simulink model "Mophong"  (R2024a)
settings: Solver=ode3  StartTime=0.0  StopTime=10  FixedStep=0.01  RelTol=1e-3
values from neighbouring files (symbols this model uses):
  A = [0,                                                                                                                                                                                                                                                                1,                                                                                                                                            ...(+395 chars)    [CacFunctionTrongSimulink_LQR.m]
  B = [                                                                                                                                                                                                                   0,                                                                                                                                                                                           ...(+27 chars)    [CacFunctionTrongSimulink_LQR.m]
  C = [1 0 0 0 0 0 ... (first row only)    [CacFunctionTrongSimulink_LQR.m]
  x1_init = 0.003    [CacFunctionTrongSimulink_LQR.m]
  x2_init = -0.0012    [CacFunctionTrongSimulink_LQR.m]
  x4_init = 0.002    [CacFunctionTrongSimulink_LQR.m]
  x5_init = -0.002    [CacFunctionTrongSimulink_LQR.m]
  x7_init = 0.002    [CacFunctionTrongSimulink_LQR.m]
  x8_init = -0.0014    [CacFunctionTrongSimulink_LQR.m]
undefined symbols (not defined in the file or in its folder): K, Lk
libraries: simulink x3
settings Model: Creator=nguye  LastModifiedBy=HP

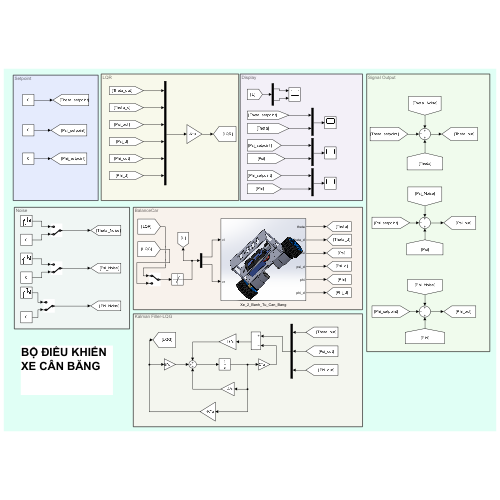
[thumbnail: Simulink's stored preview of the top-level diagram]
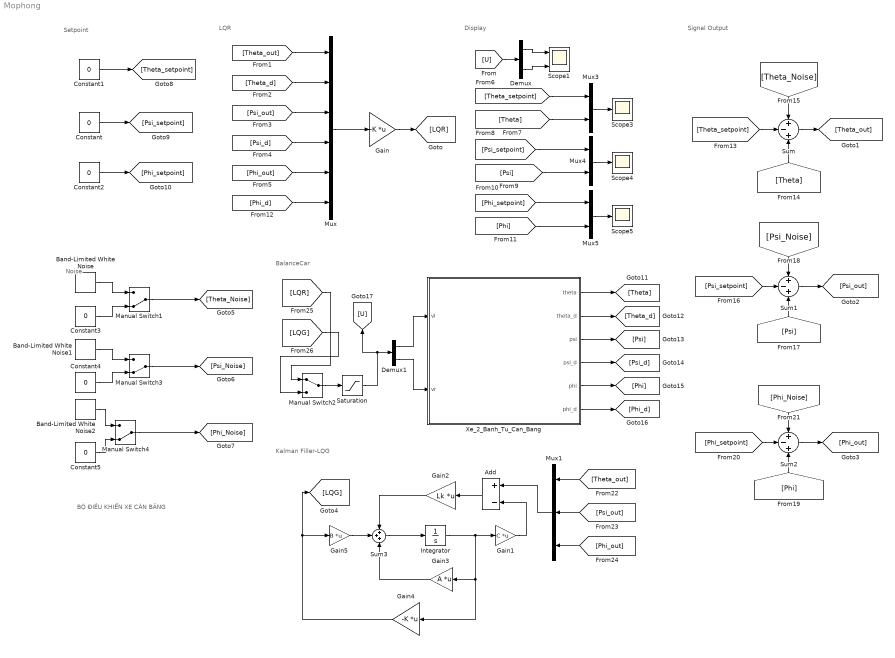
== system Mophong ==
  note: BỘ ĐIỀU KHIỂN XE CÂN BĂNG
  note: BalanceCar
  note: Setpoint
  note: LQR
  note: Display
  note: Signal Output
  note: Kalman Filler-LQG
  note: Noise
  Add : Sum  Inputs=+-
  Band-Limited White Noise : simulink/Sources/Band-Limited White Noise  Cov=[ 0.0001]  Ts=0.01  seed=[23341]
  Band-Limited White Noise1 : simulink/Sources/Band-Limited White Noise  Cov=[0.0000001]  Ts=0.01  seed=[23341]
  Band-Limited White Noise2 : simulink/Sources/Band-Limited White Noise  Cov=[0.00001]  Ts=0.01  seed=[23341]
  Constant{,1..5} (6 alike) : Constant  Value=0
  Demux : Demux  Outputs=2
  Demux1 : Demux  Outputs=2
  Gain : Gain  Gain=-K  Multiplication=Matrix(K*u)
  Gain1 : Gain  Gain=C  Multiplication=Matrix(K*u)
  Gain2 : Gain  Gain=Lk  Multiplication=Matrix(K*u)
  Gain3 : Gain  Gain=A  Multiplication=Matrix(K*u)
  Gain4 : Gain  Gain=-K  Multiplication=Matrix(K*u)
  Gain5 : Gain  Gain=B  Multiplication=Matrix(K*u)
  Integrator : Integrator
  Manual Switch1 : ManualSwitch  CurrentSetting=0
  Manual Switch2 : ManualSwitch
  Manual Switch3 : ManualSwitch  CurrentSetting=0
  Manual Switch4 : ManualSwitch  CurrentSetting=0
  Mux : Mux  Inputs=6
  Mux1 : Mux  Inputs=3
  Mux3 : Mux  Inputs=2
  Mux4 : Mux  Inputs=2
  Mux5 : Mux  Inputs=2
  Saturation : Saturate  UpperLimit=255  LowerLimit=-255
  Scope1 : Scope  NumInputPorts=2
  Scope3 : Scope
  Scope4 : Scope
  Scope5 : Scope
  Sum : Sum  Inputs=+-+
  Sum1 : Sum  Inputs=+-+
  Sum2 : Sum  Inputs=+-+
  Sum3 : Sum  Inputs=+++
  Xe_2_Banh_Tu_Can_Bang : Subsystem
      mask Display: image('BalanceCar.png');
  wires:
  Mux4/1 -> Scope4/1
  Mux3/1 -> Scope3/1
  [Phi] -> Mux5/2
  [Phi_setpoint] -> Mux5/1
  [Psi] -> Mux4/2
  [Psi_setpoint] -> Mux4/1
  [Theta] -> Mux3/2
  [U] -> Demux/1
  Demux/1 -> Scope1/1
  Demux/2 -> Scope1/2
  [Theta_out] -> Mux/1
  [Theta_d] -> Mux/2
  [Psi_out] -> Mux/3
  [Psi_d] -> Mux/4
  [Phi_out] -> Mux/5
  [Phi_d] -> Mux/6
  Mux/1 -> Gain/1
  Gain/1 -> [LQR]
  [Theta_Noise] -> Sum/1
  Sum/1 -> [Theta_out]
  Sum1/1 -> [Psi_out]
  [Psi_Noise] -> Sum1/1
  [Phi_Noise] -> Sum2/1
  Sum2/1 -> [Phi_out]
  [Theta_out] -> Mux1/1
  [Psi_out] -> Mux1/2
  Mux1/1 -> Add/1
  Add/1 -> Gain2/1
  Sum3/1 -> Integrator/1
  Gain3/1 -> Sum3/3
  Gain5/1 -> Sum3/2
  Gain2/1 -> Sum3/1
  Constant2/1 -> [Phi_setpoint]
  Constant1/1 -> [Theta_setpoint]
  Constant/1 -> [Psi_setpoint]
  [LQR] -> Manual Switch2/1
  [LQG] -> Manual Switch2/2
  Integrator/1 -> Gain1/1, Gain4/1, Gain3/1
  Xe_2_Banh_Tu_Can_Bang/1(theta) -> [Theta]
  Xe_2_Banh_Tu_Can_Bang/2(theta_d) -> [Theta_d]
  Xe_2_Banh_Tu_Can_Bang/3(psi) -> [Psi]
  Xe_2_Banh_Tu_Can_Bang/4(psi_d) -> [Psi_d]
  Xe_2_Banh_Tu_Can_Bang/5(phi) -> [Phi]
  Xe_2_Banh_Tu_Can_Bang/6(phi_d) -> [Phi_d]
  Demux1/1 -> Xe_2_Banh_Tu_Can_Bang/1(vl)
  Demux1/2 -> Xe_2_Banh_Tu_Can_Bang/2(vr)
  Mux5/1 -> Scope5/1
  [Phi_out] -> Mux1/3
  Gain4/1 -> [LQG], Gain5/1
  Band-Limited White Noise/1 -> Manual Switch1/1
  Manual Switch1/1 -> [Theta_Noise]
  Constant3/1 -> Manual Switch1/2
  Band-Limited White Noise1/1 -> Manual Switch3/1
  Constant4/1 -> Manual Switch3/2
  Manual Switch3/1 -> [Psi_Noise]
  Band-Limited White Noise2/1 -> Manual Switch4/1
  Manual Switch4/1 -> [Phi_Noise]
  Constant5/1 -> Manual Switch4/2
  Gain1/1 -> Add/2
  [Theta_setpoint] -> Mux3/1
  Manual Switch2/1 -> Saturation/1
  Saturation/1 -> Demux1/1, [U]
  [Theta] -> Sum/3
  [Theta_setpoint] -> Sum/2
  [Psi] -> Sum1/3
  [Psi_setpoint] -> Sum1/2
  [Phi] -> Sum2/3
  [Phi_setpoint] -> Sum2/2

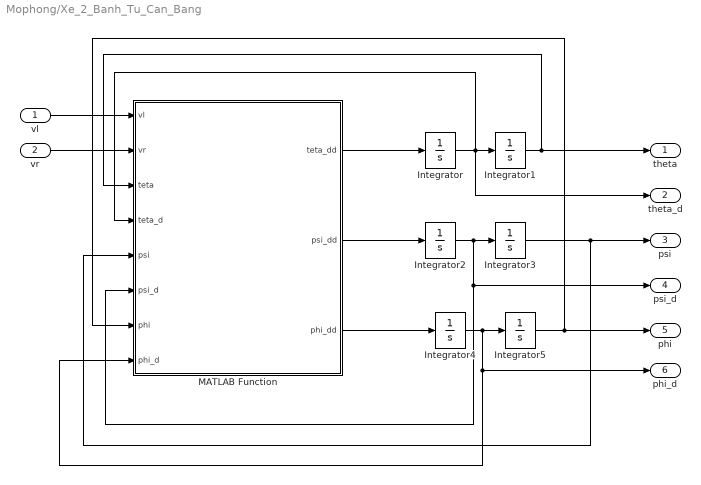
== system Mophong/Xe_2_Banh_Tu_Can_Bang ==
  vl : Inport
  vr : Inport  Port=2
  Integrator : Integrator  InitialCondition=x2_init
  Integrator1 : Integrator  InitialCondition=x1_init
  Integrator2 : Integrator  InitialCondition=x5_init
  Integrator3 : Integrator  InitialCondition=x4_init
  Integrator4 : Integrator  InitialCondition=x8_init
  Integrator5 : Integrator  InitialCondition=x7_init
  MATLAB Function : MATLAB Function  TreatAsAtomicUnit=on
  theta : Outport
  theta_d : Outport  Port=2
  psi : Outport  Port=3
  psi_d : Outport  Port=4
  phi : Outport  Port=5
  phi_d : Outport  Port=6
  wires:
  Integrator/1 -> MATLAB Function/4(teta_d), Integrator1/1, theta_d/1
  Integrator1/1 -> MATLAB Function/3(teta), theta/1
  MATLAB Function/1(teta_dd) -> Integrator/1
  Integrator3/1 -> MATLAB Function/5(psi), psi/1
  Integrator2/1 -> MATLAB Function/6(psi_d), psi_d/1, Integrator3/1
  MATLAB Function/2(psi_dd) -> Integrator2/1
  Integrator5/1 -> MATLAB Function/7(phi), phi/1
  Integrator4/1 -> MATLAB Function/8(phi_d), phi_d/1, Integrator5/1
  MATLAB Function/3(phi_dd) -> Integrator4/1
  vr/1 -> MATLAB Function/2(vr)
  vl/1 -> MATLAB Function/1(vl)

== matlab function Mophong/Xe_2_Banh_Tu_Can_Bang/MATLAB Function ==
  data: vl input; teta_dd output; vr input; teta input; teta_d input; psi input; psi_d input; phi input; phi_d input; psi_dd output; phi_dd output
function [teta_dd,psi_dd,phi_dd] = fcn(vl,vr,teta,teta_d,psi,psi_d,phi,phi_d)

%% Thông số hệ thống xe 2 bánh tự cân bằng dùng LQR
m = 0.033; %Khoi luong banh xe
M = 0.818; %Khoi luong robot
R = 0.0325; %Ban kinh ban xe
W = 0.15; %Chieu dai robot
D = 0.07; %Chieu rong robot
H = 0.095; %Chieu cao robot
L = 0.06; %khoang cach tu trong tam den truc banh xe
fw = 0.18; %He so ma sat giua banh xe voi mat phang
fm = 0.002; %he so ma sat giua dong co va robot
Jm = 0.01; %moment quan tinh cua dong co
Jw = m*R^2/2;
J_psi = 2*M*L^2/3;
J_phi = M*(W^2+D^2)/12;
Rm = 40; %Dien tro dong co DC
Kb = 0.327; %he so emf cua dong co
Kt = 0.5; %Momen xoan cua dong co DC
n = 30; %Ty so giam toc
g = 9.81; %Gia toc trong truong
alpha = (n*Kt)/Rm; beta=((n*Kt*Kb)/Rm)+fm; a =alpha;
T=0.01;

teta_dd = (J_psi*a*vl + J_psi*a*vr - 2*J_psi*beta*teta_d + 2*J_psi*beta*psi_d - 2*J_psi*fw*teta_d + L^2*M*a*vl + L^2*M*a*vr - 2*L^2*M*beta*teta_d + 2*L^2*M*beta*psi_d - 2*L^2*M*fw*teta_d - 4*Jm*fw*n^2*teta_d + L^3*M^2*R*psi_d^2*sin(psi) - 2*L*M*R*beta*teta_d*cos(psi) + 2*L*M*R*beta*psi_d*cos(psi) - L^3*M^2*R*phi_d^2*cos(psi)^2*sin(psi) - L^2*M^2*R*g*cos(psi)*sin(psi) + J_psi*L*M*R*psi_d^2*sin(psi) + 2*Jm*L*M*g*n^2*sin(psi) + L*M*R*a*vl*cos(psi) + L*M*R*a*vr*cos(psi) + 2*Jm*L^2*M*n^2*phi_d^2*cos(psi)*sin(psi) + 2*Jm*L*M*R*n^2*psi_d^2*sin(psi))/(2*J_psi*Jw + L^2*M^2*R^2 + 2*Jw*L^2*M + J_psi*M*R^2 + 2*J_psi*Jm*n^2 + 4*Jm*Jw*n^2 + 2*J_psi*R^2*m + 2*Jm*L^2*M*n^2 + 2*Jm*M*R^2*n^2 + 2*L^2*M*R^2*m + 4*Jm*R^2*m*n^2 - L^2*M^2*R^2*cos(psi)^2 + 4*Jm*L*M*R*n^2*cos(psi));
psi_dd = -(2*Jw*a*vl + 2*Jw*a*vr - 4*Jw*beta*teta_d + 4*Jw*beta*psi_d + M*R^2*a*vl + M*R^2*a*vr - 2*M*R^2*beta*teta_d + 2*M*R^2*beta*psi_d + 2*R^2*a*m*vl + 2*R^2*a*m*vr + 4*Jm*fw*n^2*teta_d - 4*R^2*beta*m*teta_d + 4*R^2*beta*m*psi_d - L*M^2*R^2*g*sin(psi) - 2*Jw*L*M*g*sin(psi) - 2*L*M*R*beta*teta_d*cos(psi) + 2*L*M*R*beta*psi_d*cos(psi) - 2*L*M*R*fw*teta_d*cos(psi) + L^2*M^2*R^2*psi_d^2*cos(psi)*sin(psi) - L^2*M^2*R^2*phi_d^2*cos(psi)*sin(psi) - 2*Jw*L^2*M*phi_d^2*cos(psi)*sin(psi) - 2*Jm*L*M*g*n^2*sin(psi) - 2*L*M*R^2*g*m*sin(psi) + L*M*R*a*vl*cos(psi) + L*M*R*a*vr*cos(psi) - 2*Jm*L^2*M*n^2*phi_d^2*cos(psi)*sin(psi) - 2*L^2*M*R^2*m*phi_d^2*cos(psi)*sin(psi) - 2*Jm*L*M*R*n^2*psi_d^2*sin(psi))/(2*J_psi*Jw + L^2*M^2*R^2 + 2*Jw*L^2*M + J_psi*M*R^2 + 2*J_psi*Jm*n^2 + 4*Jm*Jw*n^2 + 2*J_psi*R^2*m + 2*Jm*L^2*M*n^2 + 2*Jm*M*R^2*n^2 + 2*L^2*M*R^2*m + 4*Jm*R^2*m*n^2 - L^2*M^2*R^2*cos(psi)^2 + 4*Jm*L*M*R*n^2*cos(psi));
phi_dd = -(W^2*beta*phi_d + W^2*fw*phi_d + R*W*a*vl - R*W*a*vr + 4*L^2*M*R^2*psi_d*phi_d*cos(psi)*sin(psi))/(2*J_phi*R^2 + Jm*W^2 + Jm*W^2*n^2 + R^2*W^2*m + 2*L^2*M*R^2*sin(psi)^2);
